simulink model "simu_dis_MCC"  (R2025b)
settings: Solver=VariableStepAuto  StartTime=0.0  StopTime=2  FixedStep=0.04  MaxStep=0.04  RelTol=1e-3
undefined symbols (not defined in the file or in its folder): A2D, AD, B2D, BD, C2D, CD, D2D, DD

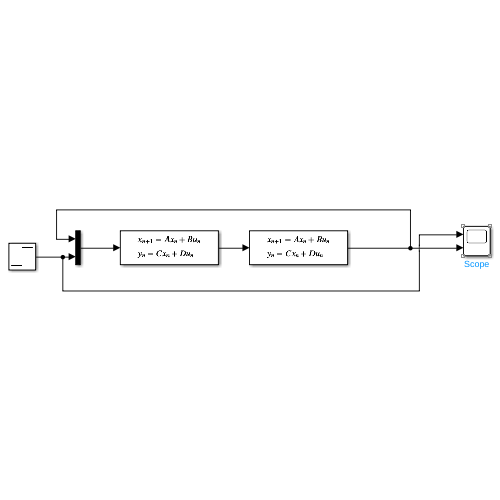
[thumbnail: Simulink's stored preview of the top-level diagram]
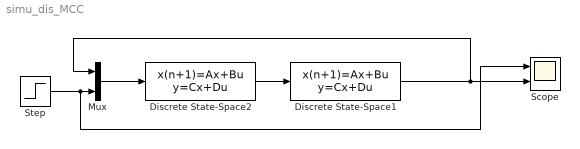
== system simu_dis_MCC ==
  Discrete State-Space1 : DiscreteStateSpace  A=A2D  B=B2D  C=C2D  D=D2D  SampleTime=0.01
  Discrete State-Space2 : DiscreteStateSpace  A=AD  B=BD  C=CD  D=DD  SampleTime=0.01
  Mux : Mux  Inputs=2
  Scope : Scope  NumInputPorts=2
      settings: ActiveDisplayYMinimum=-0.39584  ActiveDisplayYMaximum=5.2
  Step : Step  After=5  SampleTime=0.01
  wires:
  Mux/1 -> Discrete State-Space2/1
  Discrete State-Space2/1 -> Discrete State-Space1/1
  Step/1 -> Scope/1, Mux/2
  Discrete State-Space1/1 -> Mux/1, Scope/2
